simulink model "mission_s"  (R2026a)
settings: Solver=ode4  StopTime=40  FixedStep=P.dt
PostLoadFcn:
  | addpath(fileparts(get_param(bdroot, 'FileName')));
InitFcn:
  | if ~exist('P','var'), [P, ~] = ms_params(); end
  | if ~exist('PP','var'), PP = P; end
values from neighbouring files (symbols this model uses):
  P = ms_derive(P)    [ms_params.m]    (also in ms_robustness.m)
  PP = P    [run_mission_s.m]
settings Model: Creator=Mission S demo  LastModifiedBy=Mission S demo

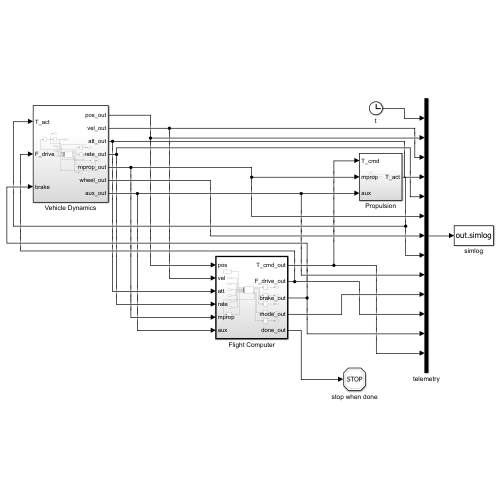
[thumbnail: Simulink's stored preview of the top-level diagram]
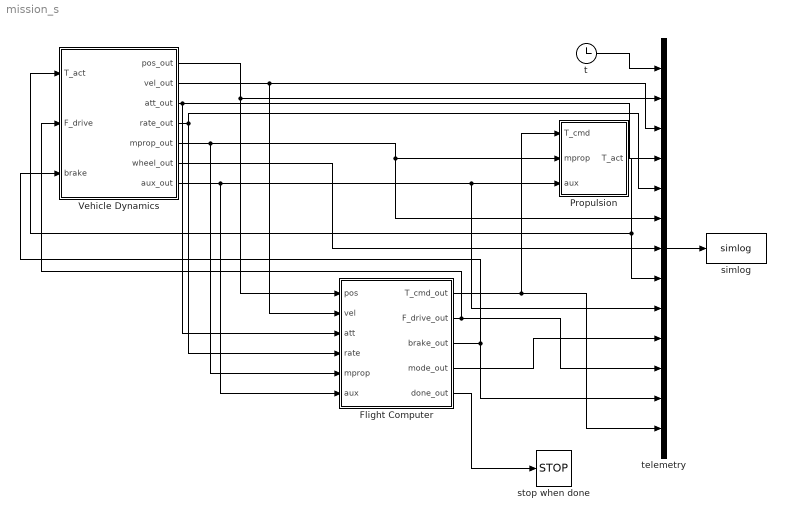
== system mission_s ==
  Flight Computer : Subsystem  TreatAsAtomicUnit=on  SystemSampleTime=P.Ts
      settings: MinAlgLoopOccurrences=on
  Propulsion : Subsystem
  Vehicle Dynamics : Subsystem
  simlog : ToWorkspace  VariableName=simlog  SampleTime=P.Ts
  stop when done : Stop
  t : Clock
  telemetry : Mux  Inputs=13
  wires:
  Vehicle Dynamics/1(pos_out) -> telemetry/2, Flight Computer/1(pos)
  Vehicle Dynamics/6(wheel_out) -> telemetry/7
  Vehicle Dynamics/2(vel_out) -> telemetry/3, Flight Computer/2(vel)
  Vehicle Dynamics/3(att_out) -> telemetry/4, Flight Computer/3(att)
  Vehicle Dynamics/4(rate_out) -> telemetry/5, Flight Computer/4(rate)
  Flight Computer/2(F_drive_out) -> Vehicle Dynamics/2(F_drive), telemetry/11
  Flight Computer/3(brake_out) -> Vehicle Dynamics/3(brake), telemetry/12
  Flight Computer/4(mode_out) -> telemetry/10
  Flight Computer/5(done_out) -> stop when done/1
  t/1 -> telemetry/1
  telemetry/1 -> simlog/1
  Propulsion/1(T_act) -> Vehicle Dynamics/1(T_act), telemetry/8
  Flight Computer/1(T_cmd_out) -> telemetry/13, Propulsion/1(T_cmd)
  Vehicle Dynamics/7(aux_out) -> telemetry/9, Propulsion/3(aux), Flight Computer/6(aux)
  Vehicle Dynamics/5(mprop_out) -> Propulsion/2(mprop), telemetry/6, Flight Computer/5(mprop)

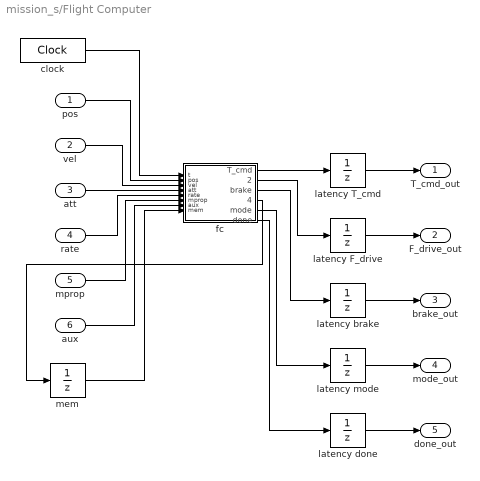
== system mission_s/Flight Computer ==
  pos : Inport
  vel : Inport  Port=2
  att : Inport  Port=3
  rate : Inport  Port=4
  mprop : Inport  Port=5
  aux : Inport  Port=6
  clock : DigitalClock  SampleTime=P.Ts
  fc : MATLAB Function  TreatAsAtomicUnit=on
  latency F_drive : UnitDelay  SampleTime=P.Ts
  latency T_cmd : UnitDelay  InitialCondition=zeros(P.n_thr,1)  SampleTime=P.Ts
  latency brake : UnitDelay  SampleTime=P.Ts
  latency done : UnitDelay  SampleTime=P.Ts
  latency mode : UnitDelay  SampleTime=P.Ts
  mem : UnitDelay  InitialCondition=P.mem0  SampleTime=P.Ts
  T_cmd_out : Outport
  F_drive_out : Outport  Port=2
  brake_out : Outport  Port=3
  mode_out : Outport  Port=4
  done_out : Outport  Port=5
  wires:
  clock/1 -> fc/1(t)
  latency T_cmd/1 -> T_cmd_out/1
  pos/1 -> fc/2(pos)
  vel/1 -> fc/3(vel)
  att/1 -> fc/4(att)
  rate/1 -> fc/5(rate)
  mprop/1 -> fc/6(mprop)
  latency mode/1 -> mode_out/1
  aux/1 -> fc/7(aux)
  mem/1 -> fc/8(mem)
  fc/1(T_cmd) -> latency T_cmd/1
  latency done/1 -> done_out/1
  fc/2(F_drive) -> latency F_drive/1
  fc/3(brake) -> latency brake/1
  fc/4(mem_out) -> mem/1
  fc/5(mode) -> latency mode/1
  fc/6(done) -> latency done/1
  latency F_drive/1 -> F_drive_out/1
  latency brake/1 -> brake_out/1

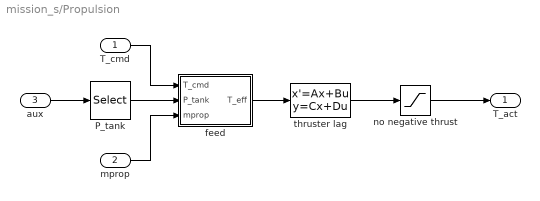
== system mission_s/Propulsion ==
  T_cmd : Inport
  mprop : Inport  Port=2
  aux : Inport  Port=3
  P_tank : Selector  InputPortWidth=14  IndexOptions=Index vector (dialog)  Indices=10  OutputSizes=1
  feed : MATLAB Function  TreatAsAtomicUnit=on
  no negative thrust : Saturate  UpperLimit=inf  LowerLimit=0
  thruster lag : StateSpace  A=-diag(1./PP.tau)  B=diag(1./PP.tau)  C=eye(PP.n_thr)  D=zeros(PP.n_thr)  InitialCondition=zeros(PP.n_thr,1)
  T_act : Outport
  wires:
  aux/1 -> P_tank/1
  T_cmd/1 -> feed/1(T_cmd)
  feed/1(T_eff) -> thruster lag/1
  P_tank/1 -> feed/2(P_tank)
  no negative thrust/1 -> T_act/1
  mprop/1 -> feed/3(mprop)
  thruster lag/1 -> no negative thrust/1

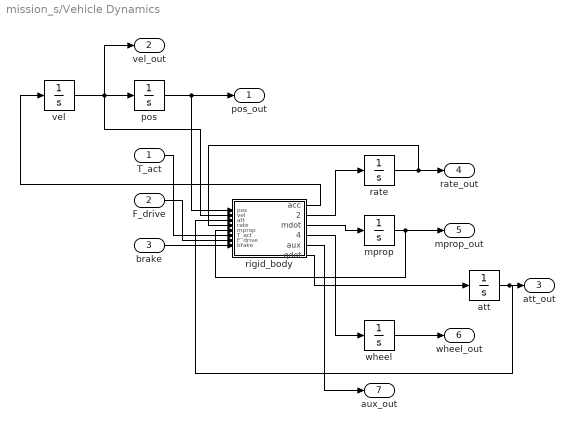
== system mission_s/Vehicle Dynamics ==
  T_act : Inport
  F_drive : Inport  Port=2
  brake : Inport  Port=3
  att : Integrator  InitialCondition=[1;0;0;0]
  mprop : Integrator  InitialCondition=[PP.m_f0; PP.m_o0]  LimitOutput=on  LowerSaturationLimit=0
  pos : Integrator  InitialCondition=PP.pos0
  rate : Integrator  InitialCondition=zeros(3,1)
  rigid_body : MATLAB Function  TreatAsAtomicUnit=on
  vel : Integrator  InitialCondition=[0;0;0]
  wheel : Integrator
  pos_out : Outport
  vel_out : Outport  Port=2
  att_out : Outport  Port=3
  rate_out : Outport  Port=4
  mprop_out : Outport  Port=5
  wheel_out : Outport  Port=6
  aux_out : Outport  Port=7
  wires:
  vel/1 -> rigid_body/2(vel), vel_out/1, pos/1
  rigid_body/2(angacc) -> rate/1
  pos/1 -> rigid_body/1(pos), pos_out/1
  T_act/1 -> rigid_body/6(T_act)
  F_drive/1 -> rigid_body/7(F_drive)
  rigid_body/1(acc) -> vel/1
  brake/1 -> rigid_body/8(brake)
  rigid_body/3(mdot) -> mprop/1
  rigid_body/4(wheel_rate) -> wheel/1
  rigid_body/5(aux) -> aux_out/1
  rate/1 -> rigid_body/4(rate), rate_out/1
  mprop/1 -> rigid_body/5(mprop), mprop_out/1
  wheel/1 -> wheel_out/1
  rigid_body/6(qdot) -> att/1
  att/1 -> rigid_body/3(att), att_out/1

== matlab function mission_s/Propulsion/feed ==
  data: T_cmd input; T_eff output; P_tank input; mprop input; PP parameter
function T_eff = feed(T_cmd, P_tank, mprop, PP)
T_eff = ms_feed(T_cmd, P_tank, mprop, PP);

== matlab function mission_s/Vehicle Dynamics/rigid_body ==
  data: pos input; acc output; vel input; att input; rate input; mprop input; T_act input; F_drive input; brake input; angacc output; mdot output; wheel_rate output; aux output; PP parameter; qdot output
function [acc, angacc, mdot, wheel_rate, aux, qdot] = rigid_body(pos, vel, att, rate, mprop, T_act, F_drive, brake, PP)
[acc, angacc, mdot, wheel_rate, aux, qdot] = ms_plant(pos, vel, att, rate, mprop, T_act, F_drive, brake, PP);

== matlab function mission_s/Flight Computer/fc ==
  data: t input; T_cmd output; pos input; vel input; att input; rate input; mprop input; aux input; mem input; F_drive output; brake output; mem_out output; mode output; done output; P parameter
function [T_cmd, F_drive, brake, mem_out, mode, done] = fc(t, pos, vel, att, rate, mprop, aux, mem, P)
[T_cmd, F_drive, brake, mem_out, mode, done] = ms_flight_computer(t, pos, vel, att, rate, mprop, aux, mem, P);
